simulink model "new"  (R2025b)
settings: Solver=ode1  StartTime=0.0  StopTime=10  FixedStep=Ts_pwm  RelTol=1e-3
values from neighbouring files (symbols this model uses):
  A = [ -Rs/L,           0,                  0 ... (first row only)    [mcb_pmsm_fsfb_f28379d_param.m]    (also in v0_pmsm_fsfb_sim_for_flipsky_.m = [; v1_0_3_sim_param_fsfc.m = [)
  B = [ 1/L,  0 ... (first row only)    [mcb_pmsm_fsfb_f28379d_param.m]    (also in v0_pmsm_fsfb_sim_for_flipsky_.m = [; v1_0_3_sim_param_fsfc.m = [)
  Bv = pmsm.B    [mcb_pmsm_foc_qep_f28379d_SIUnit_data.m]    (also in mcb_pmsm_fsfb_f28379d_param.m = 2.636e-06; v0_pmsm_fsfb_sim_for_flipsky_.m = 9.444e-05; v1_0_3_sim_param_fsfc.m = 9.444e-05)
  C = [ 1, 0, 0 ... (first row only)    [mcb_pmsm_fsfb_f28379d_param.m]    (also in v0_pmsm_fsfb_sim_for_flipsky_.m = [; v1_0_3_sim_param_fsfc.m = [)
  J = 7.061e-6    (= 7.061e-06)    [mcb_pmsm_fsfb_f28379d_param.m]    (also in v0_pmsm_fsfb_sim_for_flipsky_.m = 0.00036179; v1_0_3_sim_param_fsfc.m = 0.00036179)
  Ki = -Ka_fsfb(2)    [mcb_pmsm_foc_qep_f28379d_SIUnit_data.m]    (also in mcb_pmsm_fsfb_f28379d_param.m = -K(:, n+1:end); v0_pmsm_fsfb_sim_for_flipsky_.m = -K(:, n+1:end); v1_0_3_sim_param_fsfc.m = -K(:, n+1:end))
  Kx = K(:, 1:n)    [mcb_pmsm_fsfb_f28379d_param.m]    (also in v0_pmsm_fsfb_sim_for_flipsky_.m; v1_0_3_sim_param_fsfc.m)
  L = Ld    (= 0.0002)    [mcb_pmsm_fsfb_f28379d_param.m]    (also in v0_pmsm_fsfb_sim_for_flipsky_.m = 0.0004; v1_0_3_sim_param_fsfc.m = 0.0013)
  Lambda_m = 0.01273    [mcb_pmsm_fsfb_f28379d_param.m]    (also in v0_pmsm_fsfb_sim_for_flipsky_.m = 0.0426; v1_0_3_sim_param_fsfc.m = 0.08627)
  P = 8    [mcb_pmsm_fsfb_f28379d_param.m]    (also in v0_pmsm_fsfb_sim_for_flipsky_.m; v1_0_3_sim_param_fsfc.m)
  Pk0 = 5e-4*diag([1e-3, 1e-2, 0.2, 0.01])    [v0_pmsm_fsfb_sim_for_flipsky_.m]    (also in v1_0_3_sim_param_fsfc.m)
  Qd = 1e-4*diag([0.5, 0.5, 5, 0.5])    [v0_pmsm_fsfb_sim_for_flipsky_.m]    (also in v1_0_3_sim_param_fsfc.m)
  R = Rs    (= 0.72)    [v0_pmsm_fsfb_sim_for_flipsky_.m]    (also in v1_0_3_sim_param_fsfc.m = 0.52)
  Rc = 56.33    [v0_pmsm_fsfb_sim_for_flipsky_.m]    (also in v1_0_3_sim_param_fsfc.m = 450)
  Rs = 0.3819    [mcb_pmsm_fsfb_f28379d_param.m]    (also in v0_pmsm_fsfb_sim_for_flipsky_.m = 0.72; v1_0_3_sim_param_fsfc.m = 0.52)
  Tc = 0.001    [v0_pmsm_fsfb_sim_for_flipsky_.m]    (also in v1_0_3_sim_param_fsfc.m)
  Ts = T_pwm    (= 5e-05)    [mcb_pmsm_foc_qep_f28379d_SIUnit_data.m]    (also in v0_pmsm_fsfb_sim_for_flipsky_.m = 0.0001; v1_0_3_sim_param_fsfc.m = 0.0001)
  Ts_ov = 1e-6    (= 1e-06)    [v0_pmsm_fsfb_sim_for_flipsky_.m]    (also in v1_0_3_sim_param_fsfc.m)
  Ts_pwm = 1/20000    (= 5e-05)    [mcb_pmsm_fsfb_f28379d_param.m]    (also in v0_pmsm_fsfb_sim_for_flipsky_.m = 0.0001; v1_0_3_sim_param_fsfc.m = 0.0001)
  Vdc = 24    [mcb_pmsm_fsfb_f28379d_param.m]    (also in v0_pmsm_fsfb_sim_for_flipsky_.m = 48*sqrt(3); v1_0_3_sim_param_fsfc.m = 150*sqrt(3))
  X03 = [0; 0; 0]    [v0_pmsm_fsfb_sim_for_flipsky_.m]    (also in v1_0_3_sim_param_fsfc.m)
  X04 = 1e-2*[1; 1; 1; 0]    [v0_pmsm_fsfb_sim_for_flipsky_.m]    (also in v1_0_3_sim_param_fsfc.m)
undefined symbols (not defined in the file or in its folder): Down, Up
libraries: spsMosfetLib x6, simulink x4, spsDCVoltageSourceLib x1, spsGroundLib x1, spsPermanentMagnetSynchronousMachineLib x1, spsThreePhaseVIMeasurementLib x1, spspowerguiLib x1, eeGeneralControl x1, spsSVPWMGenerator2LevelLib x1
(part 2 of 2)

== matlab function new/Optimization/Optim_Omega_m_shifting ==
  data: Omega_m_opt output; Eff_opt output; Jc_min output; TL input; Rc parameter; Lambda_m parameter; L parameter; P parameter; Rs parameter; Tc parameter; Bv parameter; J parameter
function [Omega_m_opt, Eff_opt, Jc_min] = fcn(TL, Rc, Lambda_m, L, P, Rs, Tc, Bv, J)

Omega_m_min = 500; %rpm
Omega_m_max = 4000; %rmp

Omega_m_min = Omega_m_min*2*pi/60; %rad/s
Omega_m_max = Omega_m_max*2*pi/60; %rad/s

Omega_e_min = (P/2)*Omega_m_min*2*pi/60; %rad/s
Omega_e_max = (P/2)*Omega_m_max*2*pi/60; %rad/s

%% Method 1

% Eff_opt = 0;
% Omega_e_opt = Omega_m_max*P/2;
% for Omega_m = linspace(Omega_m_min, Omega_m_max, 1000)
%     Omega_e = Omega_m*P/2;
%      Eff_opt_calc = Calculate_Eff(Omega_e, idq, u, Rc, Lambda_m, L, P, Rs, Tc, Bv);
%      if Eff_opt_calc > Eff_opt
%          Eff_opt = Eff_opt_calc;
%          Omega_e_opt = Omega_e;
%      end
% end
%% Method 2
% Omega_m_a = Omega_m_min;
% Omega_e_a = Omega_m_a*P/2;
% 
% Omega_m_b = Omega_m_max;
% Omega_e_b = Omega_m_b*P/2;
% 
% a = Omega_e_a;
% b = Omega_e_b;
% tol = 1e-4;
% 
% for i = 1:500
%     c = (a+b)/2;
%     dEff_c = Calculate_dEff(c, idq, u, Rc, Lambda_m, L, P, Rs, Tc, Bv);
% 
%     if abs(b - a) < tol
%         break;
%     end
% 
%     if dEff_c > 0
%         a = c;
%     else
%         b = c;
%     end
% 
% end
% Compute optimal Omega_m_opt
% Omega_e_opt = (a + b) / 2;
%% Method 3
alpha = 0.75;
theta_e = 2*pi*100;
Eff_1min = 10;
Eff_1max = 100;

Omega_e = linspace(0, 0, 1000);
Eff = linspace(0, 0, 1000);
Jc = linspace(0, 0, 1000);
i = 0;
for Omega_m = linspace(Omega_m_min, Omega_m_max, 1000)
    i = i+1;
    Omega_e(i) = Omega_m*P/2;
    Eff(i) = Calculate_Eff(Omega_e(i), TL, Rc, Lambda_m, L, P, Rs, Tc, Bv, J);
    Eff_1n = (Eff(i) - Eff_1min)/(Eff_1max - Eff_1min);
    Eff_1n = 1/Eff_1n;
    t_min = theta_e/Omega_e_max;
    t_max = theta_e/Omega_e_min;
    t = theta_e/Omega_e(i);
    t_n = (t - t_min)/(t_max - t_min);
    Jc(i) = alpha*Eff_1n + (1 - alpha)*t_n;

end
[Jc_min, Jc_idx] = min(Jc);
Omega_e_opt = Omega_e(Jc_idx);
Omega_m_opt = Omega_e_opt * 2 / P;
Eff_opt = Eff(Jc_idx);


if Eff_opt < 0.2
    Eff_opt = 0.2;
elseif Eff_opt > 1
    Eff_opt = 1;
end
Eff_opt = Eff_opt*100;



%% Calculate Pin
function Eff = Calculate_Eff(Omega_e, TL, Rc, Lambda_m, L, P, Rs, Tc, Bv, J)
    
    % dt = 0.00001;
    % Omega_e_dot = (Omega_e - Omega_e_dot)/dt;
    Omega_e_dot = 0;
    id = 0;

    Te = J*Omega_e_dot*2/P + TL + Bv*Omega_e*2/P;
    % iq = Te*4/(3*P*Lambda_m);

    iq = 4*Te*(Rc^2 + (L*Omega_e)^2)/(3*P*Lambda_m*Rc^2) + (Lambda_m*Omega_e - L*id*Omega_e)/Rc;

    % Calculate P_e
    P_e = Te*Omega_e*2/P;
    
    % Calculate P_Fe
    Iod_num = Rc^2*id + Rc*L*Omega_e*iq - L*Omega_e^2*Lambda_m;
    Iod_denum = Rc^2 + (L*Omega_e)^2;
    Iod = Iod_num/Iod_denum;
    
    Ioq_num = Rc*(Rc*iq - Lambda_m*Omega_e - L*id*Omega_e);
    Ioq_denum = Iod_denum;
    Ioq = Ioq_num/Ioq_denum;
    
    factor = (3/2)*(Omega_e^2/Rc);
    term1 = L*Ioq;
    term2 = Lambda_m + L*Iod;
    
    P_Fe = factor*(term1^2 + term2^2);
    
    % Calculate P_Cu
    factor_cu = (3/2)*Rs;
    term1_cu = Iod - (Omega_e*L*Ioq/Rc);
    term2_cu = Ioq + Omega_e*(Lambda_m + L*Iod)/Rc;
    
    P_Cu = factor_cu*(term1_cu^2 + term2_cu^2);
    
    % Calculate P_s
    P_s = 0.01*(P_Cu + P_Fe + P_e);
    
    % Calculate P_m
    term1_m = 4*Bv*Omega_e^2/P^2;
    term2_m = 2*Tc*Omega_e/P;
    
    P_m = term1_m + term2_m;
    
    % Calculate P_in
    P_in = P_Cu + P_Fe + P_e;
    % Calculate Efficiency
    Eff = (P_e - P_m - P_s)/P_in;
    if Eff >= 1
        Eff = 1;
    elseif Eff <= 0.1
        Eff = 10;
    end
    Eff = 100*Eff;


% %% Calculate dEfficiency
% function dEff_dWe = Calculate_dEff(Omega_e, TL, Rc, Lambda_m, L, P, Rs, Tc, Bv, J, Omega_e_dot)
% 
%     Eff1 = Calculate_Eff(Omega_e, TL, Rc, Lambda_m, L, P, Rs, Tc, Bv, J, Omega_e_dot);
%     Eff2 = Calculate_Eff(Omega_e, TL, Rc, Lambda_m, L, P, Rs, Tc, Bv, J, Omega_e_dot);
%     dOmega_e = Omega_e - Omega_e_dot;
%     dEff_dWe = (Eff2 - Eff1)/dOmega_e;


%% Calculate Omega_e_dot

== matlab function new/SVPWM/vdq2v_alpha_beta(InvPark) ==
  data: vdq input; v_alph_beta output; theta_e input
function v_alph_beta = fcn(vdq, theta_e)


v_alph_beta = [
        cos(theta_e), -sin(theta_e);
        sin(theta_e), cos(theta_e);
    ]*vdq;
